simulink model "acf_force_control_simple"  (R2026b)
settings: Solver=ode4  StopTime=4  FixedStep=1.0000000000000001e-05
InitFcn:
  | acf_select_actuator(bdroot);
model workspace (MAT data in the model file):
  acfControlVersion = 'inertial-delivery-v8'
  acfImplementation = 'simple'
  acfLayoutVersion = 1
  p : object (value not decoded)
  pCompliant : object (value not decoded)
  pNearContact : object (value not decoded)
  pNoSprings : object (value not decoded)
  pRecommended : object (value not decoded)
symbols that are objects in the model workspace (value not decoded): p
undefined symbols (not defined in the file): DiscIntNeverNeededParam
(part 2 of 3)

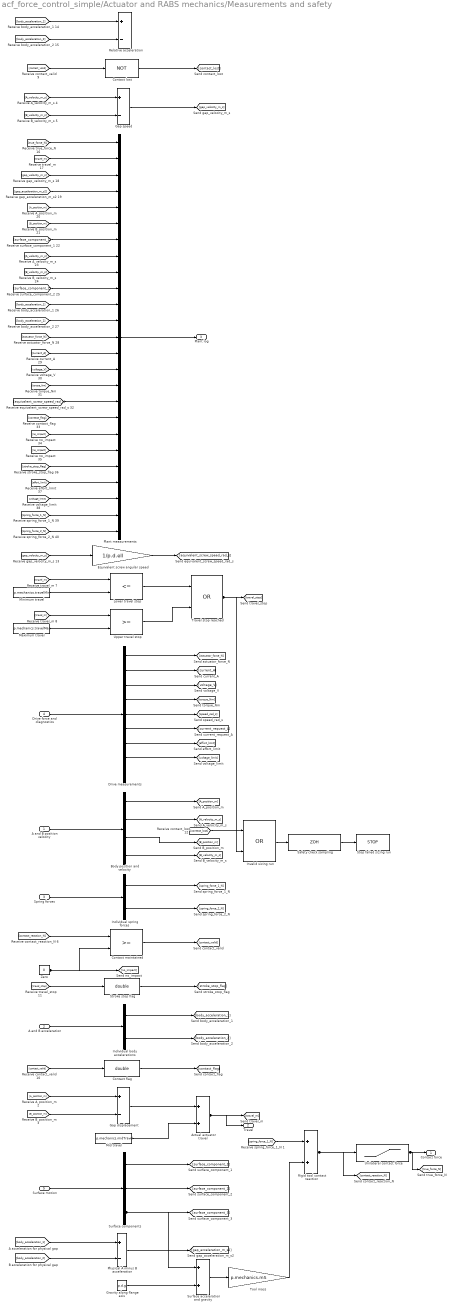
== system acf_force_control_simple/Actuator and RABS mechanics/Measurements and safety ==
  A and B position velocity : Inport
  A and B acceleration : Inport  Port=2
  Spring forces : Inport  Port=3
  Drive force and diagnostics : Inport  Port=4
  Surface motion : Inport  Port=5
  Actual actuator travel : Sum
  Body position and velocity : Demux
  Contact flag : DataTypeConversion  OutDataTypeStr=double  SaturateOnIntegerOverflow=off  RndMeth=Floor
  Contact lost : Logic  Operator=NOT  AllPortsSameDT=off  OutDataTypeStr=boolean
  Contact maintained : RelationalOperator  OutDataTypeStr=boolean  RndMeth=Simplest  InputSameDT=off
  Drive measurements : Demux  Outputs=9
  Equivalent screw angular speed : Gain  Gain=1/p.d.ell
  Gap displacement : Sum  Inputs=+-
  Gap speed : Sum  Inputs=+-
  Gravity along flange axis : Constant  Value=p.d.g
  Individual body accelerations : Demux  Outputs=2
  Individual spring forces : Demux  Outputs=2
  Invalid sizing run : Logic  Operator=OR  AllPortsSameDT=off  OutDataTypeStr=boolean
  Lower travel stop : RelationalOperator  Operator=<=  OutDataTypeStr=boolean  RndMeth=Simplest  InputSameDT=off
  Maximum travel : Constant  Value=p.mechanics.travelMax
  Mid travel : Constant  Value=p.mechanics.midTravel
  Minimum travel : Constant  Value=p.mechanics.travelMin
  Physical A minus B acceleration : Sum  Inputs=+-
  Plant measurements : Mux  Inputs=25
  Relative acceleration : Sum  Inputs=+-
  Rigid tool contact reaction : Sum
  Safety check sampling : ZeroOrderHold  SampleTime=p.sim.step
  Stop failed sizing run : Stop
  Stroke stop flag : DataTypeConversion  OutDataTypeStr=double  SaturateOnIntegerOverflow=off  RndMeth=Floor
  Surface acceleration and gravity : Sum
  Surface components : Demux  Outputs=3
  Tool mass : Gain  Gain=p.mechanics.mS
  Travel stop reached : Logic  Operator=OR  AllPortsSameDT=off  OutDataTypeStr=boolean
  Unilateral contact force : Saturate  UpperLimit=inf  LowerLimit=0
  Upper travel stop : RelationalOperator  OutDataTypeStr=boolean  RndMeth=Simplest  InputSameDT=off
  Zero : Constant  Value=0
  Contact force : Outport
  Travel : Outport  Port=2
  Plant log : Outport  Port=3
  wires:
  Tool mass/1 -> Rigid tool contact reaction/2
  Surface acceleration and gravity/1 -> Tool mass/1
  Actual actuator travel/1 -> Travel/1, [travel_m]
  [contact_lost] -> Invalid sizing run/1
  Travel stop reached/1 -> [travel_stop], Invalid sizing run/2
  Physical A minus B acceleration/1 -> [gap_acceleration_m_s2]
  Surface components/3 -> Surface acceleration and gravity/1, [surface_component_3]
  Surface components/2 -> [surface_component_2]
  Surface components/1 -> [surface_component_1]
  Mid travel/1 -> Actual actuator travel/2
  Gap displacement/1 -> Actual actuator travel/1
  Contact flag/1 -> [contact_flag]
  Individual body accelerations/2 -> [body_acceleration_2]
  Individual body accelerations/1 -> [body_acceleration_1]
  Stroke stop flag/1 -> [stroke_stop_flag]
  Rigid tool contact reaction/1 -> Unilateral contact force/1, [contact_reaction_N]
  Contact maintained/1 -> [contact_valid]
  Individual spring forces/2 -> [spring_force_2_N]
  Body position and velocity/4 -> [B_velocity_m_s]
  Drive measurements/8 -> [voltage_limit]
  Drive measurements/6 -> [current_request_A]
  [spring_force_1_N] -> Plant measurements/24
  Lower travel stop/1 -> Travel stop reached/1
  [effort_limit] -> Plant measurements/22
  Safety check sampling/1 -> Stop failed sizing run/1
  [body_acceleration_2] -> Plant measurements/12
  [stroke_stop_flag] -> Plant measurements/21
  Drive measurements/7 -> [effort_limit]
  [body_acceleration_2] -> Relative acceleration/2
  [equivalent_screw_speed_rad_s] -> Plant measurements/17
  Drive measurements/2 -> [current_A]
  [voltage_V] -> Plant measurements/15
  A and B position velocity/1 -> Body position and velocity/1
  [no_impact] -> Plant measurements/20
  [contact_flag] -> Plant measurements/18
  Body position and velocity/2 -> [A_velocity_m_s]
  [travel_stop] -> Stroke stop flag/1
  [B_velocity_m_s] -> Plant measurements/9
  [true_force_N] -> Plant measurements/1
  [no_impact] -> Plant measurements/19
  Unilateral contact force/1 -> Contact force/1, [true_force_N]
  Gap speed/1 -> [gap_velocity_m_s]
  [spring_force_2_N] -> Plant measurements/25
  [body_acceleration_1] -> Relative acceleration/1
  [B_position_m] -> Gap displacement/2
  [surface_component_1] -> Plant measurements/7
  [A_velocity_m_s] -> Plant measurements/8
  [body_acceleration_1] -> Plant measurements/11
  [surface_component_2] -> Plant measurements/10
  [travel_m] -> Lower travel stop/1
  [gap_velocity_m_s] -> Plant measurements/3
  [torque_Nm] -> Plant measurements/16
  [A_velocity_m_s] -> Gap speed/1
  Body position and velocity/3 -> [B_position_m]
  [voltage_limit] -> Plant measurements/23
  [spring_force_1_N] -> Rigid tool contact reaction/1
  [B_position_m] -> Plant measurements/6
  [travel_m] -> Plant measurements/2
  [contact_valid] -> Contact lost/1
  [B_velocity_m_s] -> Gap speed/2
  [gap_acceleration_m_s2] -> Plant measurements/4
  Zero/1 -> [no_impact], Contact maintained/2
  Maximum travel/1 -> Upper travel stop/2
  [current_A] -> Plant measurements/14
  Drive measurements/1 -> [actuator_force_N]
  [A_position_m] -> Plant measurements/5
  Minimum travel/1 -> Lower travel stop/2
  [gap_velocity_m_s] -> Equivalent screw angular speed/1
  [travel_m] -> Upper travel stop/1
  Drive force and diagnostics/1 -> Drive measurements/1
  Spring forces/1 -> Individual spring forces/1
  Invalid sizing run/1 -> Safety check sampling/1
  Gravity along flange axis/1 -> Surface acceleration and gravity/2
  [contact_reaction_N] -> Contact maintained/1
  [actuator_force_N] -> Plant measurements/13
  A and B acceleration/1 -> Individual body accelerations/1
  [contact_valid] -> Contact flag/1
  [A_position_m] -> Gap displacement/1
  Surface motion/1 -> Surface components/1
  [body_acceleration_1] -> Physical A minus B acceleration/1
  [body_acceleration_2] -> Physical A minus B acceleration/2
  Contact lost/1 -> [contact_lost]
  Plant measurements/1 -> Plant log/1
  Equivalent screw angular speed/1 -> [equivalent_screw_speed_rad_s]
  Upper travel stop/1 -> Travel stop reached/2
  Individual spring forces/1 -> [spring_force_1_N]
  Drive measurements/5 -> [speed_rad_s]
  Body position and velocity/1 -> [A_position_m]
  Drive measurements/3 -> [voltage_V]
  Drive measurements/4 -> [torque_Nm]

== system acf_force_control_simple/Actuator and RABS mechanics/R to A spring and damper ==
  A position velocity : Inport
  R position velocity : Inport  Port=2
  Rigid reaction : Inport  Port=3
  Compliant or rigid link : VariantSource  VariantControlMode=label  LabelModeActiveChoice=Rigid  VariantControls={Compliant, Rigid}
  Damping : Gain  Gain=p.mechanics.c2
  Endpoint difference : Sum  Inputs=+-
  Preload : Constant  Value=p.d.q20
  Spring and damper force : Sum  Inputs=+++
  Spring displacement and relative velocity : Demux  Outputs=2
  Stiffness : Gain  Gain=p.mechanics.k2
  Spring force : Outport
  wires:
  Compliant or rigid link/1 -> Spring force/1
  Rigid reaction/1 -> Compliant or rigid link/2
  Spring and damper force/1 -> Compliant or rigid link/1
  Preload/1 -> Spring and damper force/1
  Spring displacement and relative velocity/1 -> Stiffness/1
  Spring displacement and relative velocity/2 -> Damping/1
  Endpoint difference/1 -> Spring displacement and relative velocity/1
  Damping/1 -> Spring and damper force/3
  Stiffness/1 -> Spring and damper force/2
  R position velocity/1 -> Endpoint difference/2
  A position velocity/1 -> Endpoint difference/1

== system acf_force_control_simple/Contact force measurement/Contact force reconstruction ==
  raw_cell_error_N : Inport
  Cell error to deviation : Gain  Gain=-1
  Compensated axial reaction : Sum
  Compensated lateral reaction : Sum
  Downstream X inertia : Gain  Gain=p.sensor.distalMass_model_kg
  Downstream Z inertia : Gain  Gain=p.sensor.distalMass_model_kg
  Tared axial cell force : Bias  Bias=p.force.reference  SaturateOnIntegerOverflow=off
  axial_contact_N : Outport
  lateral_contact_N : Outport  Port=2
  tag scope: inertial_axial_contact_N=global, inertial_lateral_contact_N=global
  wires:
  Compensated lateral reaction/1 -> lateral_contact_N/1, [inertial_lateral_contact_N]
  Cell error to deviation/1 -> Tared axial cell force/1
  Compensated axial reaction/1 -> axial_contact_N/1, [inertial_axial_contact_N]
  [measured_S_acceleration_z] -> Downstream Z inertia/1
  Downstream X inertia/1 -> Compensated lateral reaction/2
  Tared axial cell force/1 -> Compensated axial reaction/1
  [measured_lateral_contact_N] -> Compensated lateral reaction/1
  Downstream Z inertia/1 -> Compensated axial reaction/2
  raw_cell_error_N/1 -> Cell error to deviation/1
  [measured_S_acceleration_x] -> Downstream X inertia/1

== system acf_force_control_simple/Contact force measurement/Head motion estimator ==
  measured_head_position_m : Inport
  Causal motion measurements : Mux  Inputs=3
  Estimated head travel : Bias  Bias=p.mechanics.midTravel+p.d.u0  SaturateOnIntegerOverflow=off
  Fresh 10 kHz position frame : ZeroOrderHold  SampleTime=p.force.sampleTime
  Fresh 10 kHz robot acceleration frame : ZeroOrderHold  SampleTime=p.force.sampleTime
  Fresh 10 kHz robot velocity frame : ZeroOrderHold  SampleTime=p.force.sampleTime
  Head gap and velocity observer : DiscreteStateSpace  A=p.d.toolMotionObserver.A  B=p.d.toolMotionObserver.B  C=p.d.toolMotionObserver.C  D=p.d.toolMotionObserver.D  InitialCondition=zeros(2,1)  SampleTime=p.force.sampleTime
  Head gap coordinate sign : Gain  Gain=-1
  Head gap displacement : Selector  InputPortWidth=2  IndexOptions=Index vector (dialog)  Indices=1  OutputSizes=1
  Head gap velocity : Selector  InputPortWidth=2  IndexOptions=Index vector (dialog)  Indices=2  OutputSizes=1
  Measured head coordinate deviation : Bias  Bias=p.d.positionMeasurementBias  SaturateOnIntegerOverflow=off
  Position common AA and EMA : DiscreteTransferFcn  Numerator=p.d.acquisition.responses.position.numerator  Denominator=p.d.acquisition.responses.position.denominator  InitialStates=(0)*p.d.acquisition.responses.position.steadyStatePerUnitInput  SampleTime=p.sensor.sampleTime
  Robot acceleration common AA and EMA : DiscreteTransferFcn  Numerator=p.d.acquisition.responses.frame.numerator  Denominator=p.d.acquisition.responses.frame.denominator  InitialStates=(0)*p.d.acquisition.responses.frame.steadyStatePerUnitInput  SampleTime=p.sensor.sampleTime
  Robot acceleration frame matching delay : Delay  DelayLength=p.d.acquisition.frameDelaySamples  InitialCondition=0  SampleTime=p.sensor.sampleTime
  Robot velocity common AA and EMA : DiscreteTransferFcn  Numerator=p.d.acquisition.responses.frame.numerator  Denominator=p.d.acquisition.responses.frame.denominator  InitialStates=(0)*p.d.acquisition.responses.frame.steadyStatePerUnitInput  SampleTime=p.sensor.sampleTime
  Robot velocity frame matching delay : Delay  DelayLength=p.d.acquisition.frameDelaySamples  InitialCondition=0  SampleTime=p.sensor.sampleTime
  head_gap_velocity_m_s : Outport
  estimated_head_travel_m : Outport  Port=2
  tag scope: inertial_head_motion_states=global, inertial_robot_acceleration_aligned=global, inertial_robot_velocity_aligned=global
  wires:
  Head gap displacement/1 -> Estimated head travel/1
  Head gap and velocity observer/1 -> [inertial_head_motion_states], Head gap velocity/1, Head gap displacement/1
  Causal motion measurements/1 -> Head gap and velocity observer/1
  Fresh 10 kHz robot acceleration frame/1 -> Causal motion measurements/2, [inertial_robot_acceleration_aligned]
  measured_head_position_m/1 -> Measured head coordinate deviation/1
  Measured head coordinate deviation/1 -> Head gap coordinate sign/1
  Robot velocity frame matching delay/1 -> Fresh 10 kHz robot velocity frame/1
  Robot velocity common AA and EMA/1 -> Robot velocity frame matching delay/1
  Robot acceleration common AA and EMA/1 -> Robot acceleration frame matching delay/1
  Estimated head travel/1 -> estimated_head_travel_m/1
  Head gap coordinate sign/1 -> Position common AA and EMA/1
  Robot acceleration frame matching delay/1 -> Fresh 10 kHz robot acceleration frame/1
  Position common AA and EMA/1 -> Fresh 10 kHz position frame/1
  Fresh 10 kHz robot velocity frame/1 -> [inertial_robot_velocity_aligned]
  [command_based_robot_velocity] -> Robot velocity common AA and EMA/1
  [command_based_robot_acceleration] -> Robot acceleration common AA and EMA/1
  Fresh 10 kHz position frame/1 -> Causal motion measurements/1
  Head gap velocity/1 -> head_gap_velocity_m_s/1
  [measured_S_acceleration_z] -> Causal motion measurements/3

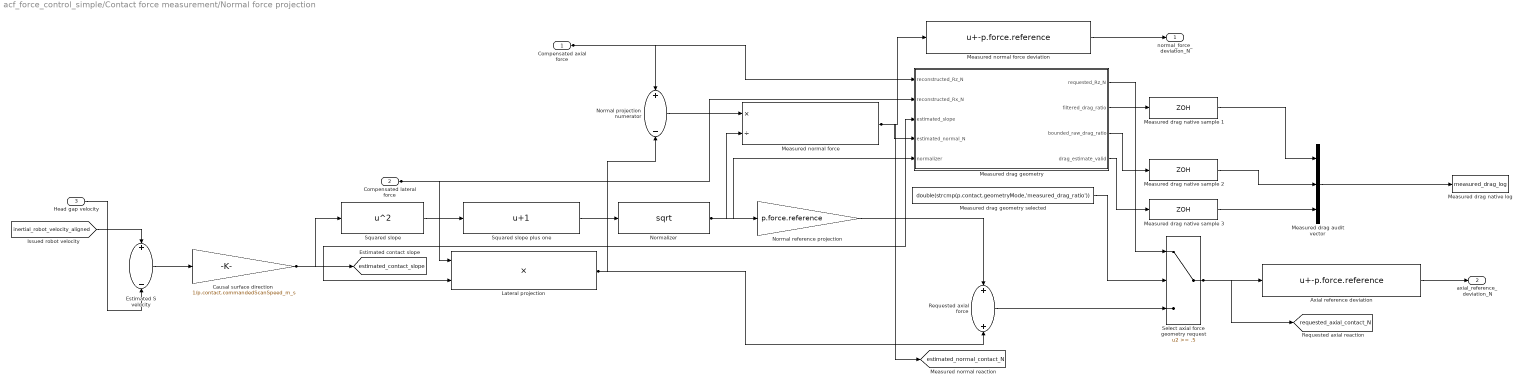
== system acf_force_control_simple/Contact force measurement/Normal force projection ==
  Compensated axial force : Inport
  Compensated lateral force : Inport  Port=2
  Head gap velocity : Inport  Port=3
  Axial reference deviation : Bias  Bias=-p.force.reference  SaturateOnIntegerOverflow=off
  Causal surface direction : Gain  Gain=1/p.contact.commandedScanSpeed_m_s
  Estimated S velocity : Sum  Inputs=+-
  Lateral projection : Product  Inputs=**
  Measured drag audit vector : Mux  Inputs=3
  Measured drag geometry : Subsystem
  Measured drag geometry selected : Constant  Value=double(strcmp(p.contact.geometryMode,'measured_drag_ratio'))
  Measured drag native log : ToWorkspace  VariableName=measured_drag_log  SaveFormat=Timeseries  SampleTime=-1
  Measured drag native sample 1 : ZeroOrderHold  SampleTime=p.sim.step
  Measured drag native sample 2 : ZeroOrderHold  SampleTime=p.sim.step
  Measured drag native sample 3 : ZeroOrderHold  SampleTime=p.sim.step
  Measured normal force : Product  Inputs=*/
  Measured normal force deviation : Bias  Bias=-p.force.reference  SaturateOnIntegerOverflow=off
  Normal projection numerator : Sum  Inputs=+-
  Normal reference projection : Gain  Gain=p.force.reference
  Normalizer : Math  Operator=sqrt
  Requested axial force : Sum
  Select axial force geometry request : Switch  Threshold=.5  SaturateOnIntegerOverflow=off  InputSameDT=off
  Squared slope : Math  Operator=square
  Squared slope plus one : Bias  Bias=1  SaturateOnIntegerOverflow=off
  normal_force_deviation_N : Outport
  axial_reference_deviation_N : Outport  Port=2
  tag scope: estimated_contact_slope=global, estimated_normal_contact_N=global, requested_axial_contact_N=global
  wires:
  Measured drag audit vector/1 -> Measured drag native log/1
  Measured drag native sample 2/1 -> Measured drag audit vector/2
  Axial reference deviation/1 -> axial_reference_deviation_N/1
  Requested axial force/1 -> Select axial force geometry request/3
  Measured drag geometry/4(drag_estimate_valid) -> Measured drag native sample 3/1
  Measured drag geometry/3(bounded_raw_drag_ratio) -> Measured drag native sample 2/1
  Measured drag geometry/2(filtered_drag_ratio) -> Measured drag native sample 1/1
  Measured drag geometry/1(requested_Rz_N) -> Select axial force geometry request/1
  Measured normal force deviation/1 -> normal_force_deviation_N/1
  Head gap velocity/1 -> Estimated S velocity/2
  [inertial_robot_velocity_aligned] -> Estimated S velocity/1
  Squared slope/1 -> Squared slope plus one/1
  Normalizer/1 -> Measured normal force/2, Normal reference projection/1, Measured drag geometry/5(normalizer)
  Causal surface direction/1 -> Squared slope/1, [estimated_contact_slope], Lateral projection/2, Measured drag geometry/3(estimated_slope)
  Measured drag geometry selected/1 -> Select axial force geometry request/2
  Normal projection numerator/1 -> Measured normal force/1
  Measured drag native sample 1/1 -> Measured drag audit vector/1
  Compensated lateral force/1 -> Lateral projection/1, Measured drag geometry/2(reconstructed_Rx_N)
  Compensated axial force/1 -> Normal projection numerator/1, Measured drag geometry/1(reconstructed_Rz_N)
  Select axial force geometry request/1 -> Axial reference deviation/1, [requested_axial_contact_N]
  Squared slope plus one/1 -> Normalizer/1
  Estimated S velocity/1 -> Causal surface direction/1
  Measured normal force/1 -> Measured normal force deviation/1, [estimated_normal_contact_N], Measured drag geometry/4(estimated_normal_N)
  Lateral projection/1 -> Normal projection numerator/2, Requested axial force/2
  Measured drag native sample 3/1 -> Measured drag audit vector/3
  Normal reference projection/1 -> Requested axial force/1

== system acf_force_control_simple/Force controller/Coil PI and PID ==
  error_N : Inport
  measured_travel_m : Inport  Port=2
  Current limits : Saturate  UpperLimit=p.coil.peakCurrent  LowerLimit=-p.coil.peakCurrent
  Current saturation error : Sum  Inputs=+-
  Flat holding current : Constant  Value=p.d.coilHoldingCurrentCommand_A
  Integral anti windup : Gain  Gain=-p.force.antiWindupRate/p.inertial.forceKi
  Lower spring inverse feedforward : Subsystem
  Measured motion feedforward : Subsystem
  Normal force PI and PID : Subsystem
  Optional structural-mode current notch : DiscreteTransferFcn  Numerator=p.d.currentNotch.numerator  Denominator=p.d.currentNotch.denominator  InitialStates=p.d.currentNotch.initialStates  SampleTime=p.force.sampleTime
  PI PID and feedforward current : Sum  Inputs=++++++
  command : Outport
  estimated_travel_m : Outport  Port=2
  estimated_force_error_N : Outport  Port=3
  wires:
  Current saturation error/1 -> Integral anti windup/1
  Current limits/1 -> command/1, Current saturation error/1
  PI PID and feedforward current/1 -> Optional structural-mode current notch/1
  Measured motion feedforward/3(friction_current_A) -> PI PID and feedforward current/5
  Measured motion feedforward/1(acceleration_current_A) -> PI PID and feedforward current/3
  Flat holding current/1 -> PI PID and feedforward current/1
  Optional structural-mode current notch/1 -> Current limits/1, Current saturation error/2
  Lower spring inverse feedforward/1(extra_current_A) -> PI PID and feedforward current/6
  Measured motion feedforward/2(geometry_current_A) -> PI PID and feedforward current/4
  Normal force PI and PID/1(feedback_current_A) -> PI PID and feedforward current/2
  error_N/1 -> Normal force PI and PID/1(error_N), estimated_force_error_N/1
  Integral anti windup/1 -> Normal force PI and PID/2(anti_windup)
  measured_travel_m/1 -> estimated_travel_m/1

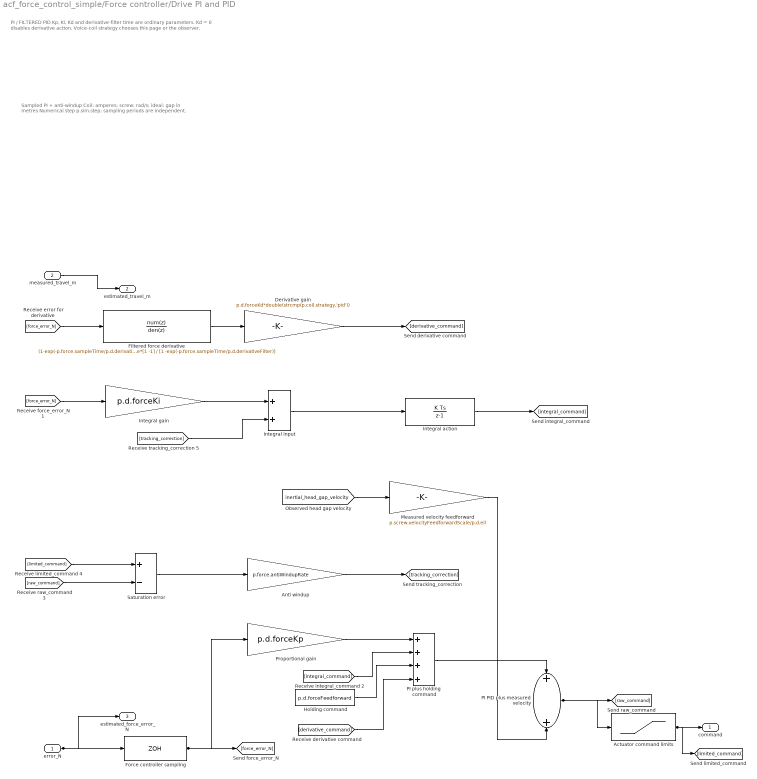
== system acf_force_control_simple/Force controller/Drive PI and PID ==
  note: Sampled PI + anti-windup
      | Coil: amperes; screw: rad/s; ideal: gap in metres
      | Numerical step p.sim.step; sampling periods are independent.
  note: PI / FILTERED PID
      | Kp, Ki, Kd and derivative-filter time are ordinary parameters.
      | Kd = 0 disables derivative action. Voice-coil strategy chooses this page or the observer.
  error_N : Inport
  measured_travel_m : Inport  Port=2
  Actuator command limits : Saturate  UpperLimit=p.d.commandMax  LowerLimit=p.d.commandMin
  Anti windup : Gain  Gain=p.force.antiWindupRate
  Derivative gain : Gain  Gain=p.d.forceKd*double(strcmp(p.coil.strategy,'pid'))
  Filtered force derivative : DiscreteTransferFcn  Numerator=(1-exp(-p.force.sampleTime/p.d.derivativeFilter))/p.force.sampleTime*[1 -1]  Denominator=[1 -exp(-p.force.sampleTime/p.d.derivativeFilter)]  SampleTime=p.force.sampleTime
  Force controller sampling : ZeroOrderHold  SampleTime=p.force.sampleTime
  Holding command : Constant  Value=p.d.forceFeedforward
  Integral action : DiscreteIntegrator  SampleTime=p.force.sampleTime  ICPrevOutput=DiscIntNeverNeededParam  ICPrevScaledInput=DiscIntNeverNeededParam
  Integral gain : Gain  Gain=p.d.forceKi
  Integral input : Sum
  Measured velocity feedforward : Gain  Gain=p.screw.velocityFeedforwardScale/p.d.ell
  PI PID plus measured velocity : Sum
  PI plus holding command : Sum  Inputs=++++
  Proportional gain : Gain  Gain=p.d.forceKp
  Saturation error : Sum  Inputs=+-
  command : Outport
  estimated_travel_m : Outport  Port=2
  estimated_force_error_N : Outport  Port=3
  wires:
  PI plus holding command/1 -> PI PID plus measured velocity/1
  [derivative_command] -> PI plus holding command/4
  Holding command/1 -> PI plus holding command/3
  [integral_command] -> PI plus holding command/2
  Proportional gain/1 -> PI plus holding command/1
  Anti windup/1 -> [tracking_correction]
  [inertial_head_gap_velocity] -> Measured velocity feedforward/1
  Filtered force derivative/1 -> Derivative gain/1
  [tracking_correction] -> Integral input/2
  Derivative gain/1 -> [derivative_command]
  Actuator command limits/1 -> [limited_command], command/1
  [force_error_N] -> Integral gain/1
  PI PID plus measured velocity/1 -> Actuator command limits/1, [raw_command]
  Integral action/1 -> [integral_command]
  measured_travel_m/1 -> estimated_travel_m/1
  [limited_command] -> Saturation error/1
  Saturation error/1 -> Anti windup/1
  [raw_command] -> Saturation error/2
  [force_error_N] -> Filtered force derivative/1
  error_N/1 -> estimated_force_error_N/1, Force controller sampling/1
  Integral gain/1 -> Integral input/1
  Force controller sampling/1 -> Proportional gain/1, [force_error_N]
  Measured velocity feedforward/1 -> PI PID plus measured velocity/2
  Integral input/1 -> Integral action/1

== system acf_force_control_simple/Force controller/Screw normal PI and PID ==
  error_N : Inport
  measured_travel_m : Inport  Port=2
  Current limits : Saturate  UpperLimit=p.screw.peakCurrent  LowerLimit=-p.screw.peakCurrent
  Current saturation error : Sum  Inputs=+-
  Flat holding current : Constant  Value=p.d.screwHoldingCurrentCommand_A
  Integral anti windup : Gain  Gain=-p.force.antiWindupRate/p.screw.currentForceKi
  Lower spring inverse feedforward : Subsystem
  Measured motion feedforward : Subsystem
  Normal force PI and PID : Subsystem
  Optional structural-mode current notch : DiscreteTransferFcn  Numerator=p.d.screwCurrentNotch.numerator  Denominator=p.d.screwCurrentNotch.denominator  InitialStates=p.d.screwCurrentNotch.initialStates  SampleTime=p.force.sampleTime
  PI PID and feedforward current : Sum  Inputs=++++++
  command : Outport
  estimated_travel_m : Outport  Port=2
  estimated_force_error_N : Outport  Port=3
  wires:
  Optional structural-mode current notch/1 -> Current limits/1, Current saturation error/2
  PI PID and feedforward current/1 -> Optional structural-mode current notch/1
  Current limits/1 -> command/1, Current saturation error/1
  Lower spring inverse feedforward/1(extra_current_A) -> PI PID and feedforward current/6
  Current saturation error/1 -> Integral anti windup/1
  Measured motion feedforward/3(friction_current_A) -> PI PID and feedforward current/5
  Measured motion feedforward/2(geometry_current_A) -> PI PID and feedforward current/4
  Integral anti windup/1 -> Normal force PI and PID/2(anti_windup)
  Measured motion feedforward/1(acceleration_current_A) -> PI PID and feedforward current/3
  Flat holding current/1 -> PI PID and feedforward current/1
  Normal force PI and PID/1(feedback_current_A) -> PI PID and feedforward current/2
  error_N/1 -> estimated_force_error_N/1, Normal force PI and PID/1(error_N)
  measured_travel_m/1 -> estimated_travel_m/1

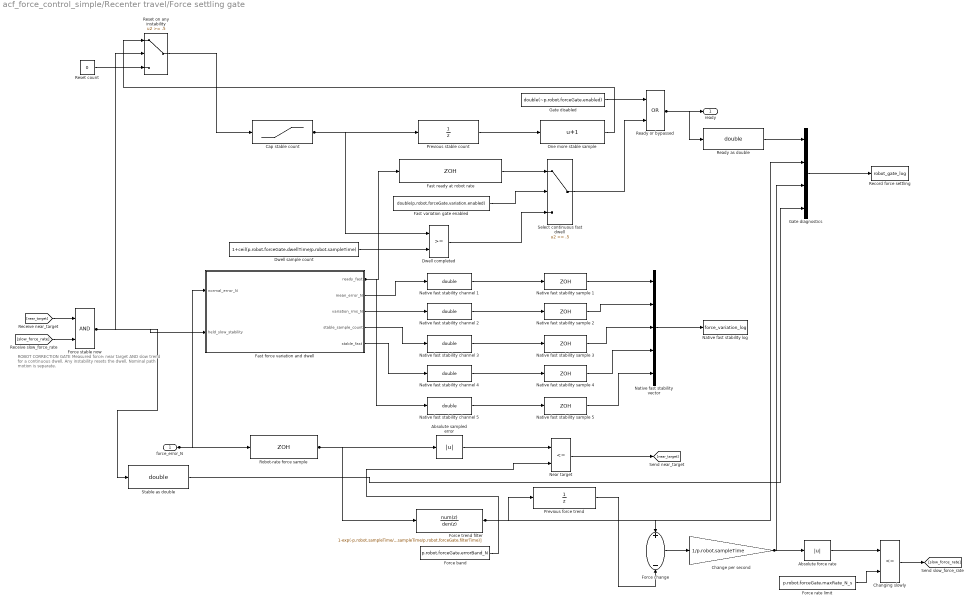
== system acf_force_control_simple/Recenter travel/Force settling gate ==
  note: ROBOT CORRECTION GATE
      | Measured force: near target AND slow trend for a continuous dwell.
      | Any instability resets the dwell. Nominal path motion is separate.
  force_error_N : Inport
  Absolute force rate : Abs  SaturateOnIntegerOverflow=off
  Absolute sampled error : Abs  SaturateOnIntegerOverflow=off
  Cap stable count : Saturate  UpperLimit=1+ceil(p.robot.forceGate.dwellTime/p.robot.sampleTime)  LowerLimit=0
  Change per second : Gain  Gain=1/p.robot.sampleTime
  Changing slowly : RelationalOperator  Operator=<=  OutDataTypeStr=boolean  RndMeth=Simplest  InputSameDT=off
  Dwell completed : RelationalOperator  OutDataTypeStr=boolean  RndMeth=Simplest  InputSameDT=off
  Dwell sample count : Constant  Value=1+ceil(p.robot.forceGate.dwellTime/p.robot.sampleTime)
  Fast force variation and dwell : Subsystem
  Fast ready at robot rate : ZeroOrderHold  SampleTime=p.robot.sampleTime
  Fast variation gate enabled : Constant  Value=double(p.robot.forceGate.variation.enabled)
  Force band : Constant  Value=p.robot.forceGate.errorBand_N
  Force change : Sum  Inputs=+-
  Force rate limit : Constant  Value=p.robot.forceGate.maxRate_N_s
  Force stable now : Logic  AllPortsSameDT=off  OutDataTypeStr=boolean
  Force trend filter : DiscreteTransferFcn  Numerator=1-exp(-p.robot.sampleTime/p.robot.forceGate.filterTime)  Denominator=[1 -exp(-p.robot.sampleTime/p.robot.forceGate.filterTime)]  SampleTime=p.robot.sampleTime
  Gate diagnostics : Mux
  Gate disabled : Constant  Value=double(~p.robot.forceGate.enabled)
  Native fast stability channel {1..5} (5 alike) : DataTypeConversion  OutDataTypeStr=double  SaturateOnIntegerOverflow=off  RndMeth=Floor
  Native fast stability log : ToWorkspace  VariableName=force_variation_log  SaveFormat=Timeseries  SampleTime=-1
  Native fast stability sample {1..5} (5 alike) : ZeroOrderHold  SampleTime=p.sim.step
  Native fast stability vector : Mux  Inputs=5
  Near target : RelationalOperator  Operator=<=  OutDataTypeStr=boolean  RndMeth=Simplest  InputSameDT=off
  One more stable sample : Bias  Bias=1  SaturateOnIntegerOverflow=off
  Previous force trend : UnitDelay  SampleTime=p.robot.sampleTime
  Previous stable count : UnitDelay  SampleTime=p.robot.sampleTime
  Ready as double : DataTypeConversion  OutDataTypeStr=double  SaturateOnIntegerOverflow=off  RndMeth=Floor
  Ready or bypassed : Logic  Operator=OR  AllPortsSameDT=off  OutDataTypeStr=boolean
  Record force settling : ToWorkspace  VariableName=robot_gate_log  SaveFormat=Timeseries  SampleTime=p.robot.sampleTime
  Reset count : Constant  Value=0
  Reset on any instability : Switch  Threshold=.5  SaturateOnIntegerOverflow=off  InputSameDT=off
  Robot-rate force sample : ZeroOrderHold  SampleTime=p.robot.sampleTime
  Select continuous fast dwell : Switch  Threshold=.5  SaturateOnIntegerOverflow=off  InputSameDT=off
  Stable as double : DataTypeConversion  OutDataTypeStr=double  SaturateOnIntegerOverflow=off  RndMeth=Floor
  ready : Outport
  wires:
  Force rate limit/1 -> Changing slowly/2
  Changing slowly/1 -> [slow_force_rate]
  Gate diagnostics/1 -> Record force settling/1
  Native fast stability vector/1 -> Native fast stability log/1
  Ready as double/1 -> Gate diagnostics/1
  Previous force trend/1 -> Force change/2
  Native fast stability sample 4/1 -> Native fast stability vector/4
  Native fast stability sample 1/1 -> Native fast stability vector/1
  Select continuous fast dwell/1 -> Ready or bypassed/2
  Fast force variation and dwell/1(ready_fast) -> Native fast stability channel 5/1, Fast ready at robot rate/1
  [slow_force_rate] -> Force stable now/2
  Force change/1 -> Change per second/1
  Native fast stability channel 4/1 -> Native fast stability sample 4/1
  Dwell sample count/1 -> Dwell completed/2
  Absolute force rate/1 -> Changing slowly/1
  Ready or bypassed/1 -> Ready as double/1, ready/1
  Reset on any instability/1 -> Cap stable count/1
  Native fast stability sample 2/1 -> Native fast stability vector/2
  Cap stable count/1 -> Dwell completed/1, Previous stable count/1
  Stable as double/1 -> Gate diagnostics/4
  Force trend filter/1 -> Previous force trend/1, Force change/1, Gate diagnostics/2
  Gate disabled/1 -> Ready or bypassed/1
  Fast force variation and dwell/3(variation_rms_N) -> Native fast stability channel 2/1
  [near_target] -> Force stable now/1
  Change per second/1 -> Gate diagnostics/3, Absolute force rate/1
  Near target/1 -> [near_target]
  Native fast stability sample 3/1 -> Native fast stability vector/3
  Fast force variation and dwell/5(stable_fast) -> Native fast stability channel 4/1
  Fast force variation and dwell/4(stable_sample_count) -> Native fast stability channel 3/1
  Force stable now/1 -> Stable as double/1, Reset on any instability/2, Fast force variation and dwell/2(held_slow_stability)
  Previous stable count/1 -> One more stable sample/1
  Fast variation gate enabled/1 -> Select continuous fast dwell/2
  Fast ready at robot rate/1 -> Select continuous fast dwell/1
  Dwell completed/1 -> Select continuous fast dwell/3
  Native fast stability channel 3/1 -> Native fast stability sample 3/1
  Native fast stability channel 1/1 -> Native fast stability sample 1/1
  force_error_N/1 -> Fast force variation and dwell/1(normal_error_N), Robot-rate force sample/1
  Native fast stability channel 2/1 -> Native fast stability sample 2/1
  Native fast stability channel 5/1 -> Native fast stability sample 5/1
  Reset count/1 -> Reset on any instability/3
  Robot-rate force sample/1 -> Force trend filter/1, Absolute sampled error/1
  Force band/1 -> Near target/2
  Native fast stability sample 5/1 -> Native fast stability vector/5
  Fast force variation and dwell/2(mean_error_N) -> Native fast stability channel 1/1
  Absolute sampled error/1 -> Near target/1
  One more stable sample/1 -> Reset on any instability/1

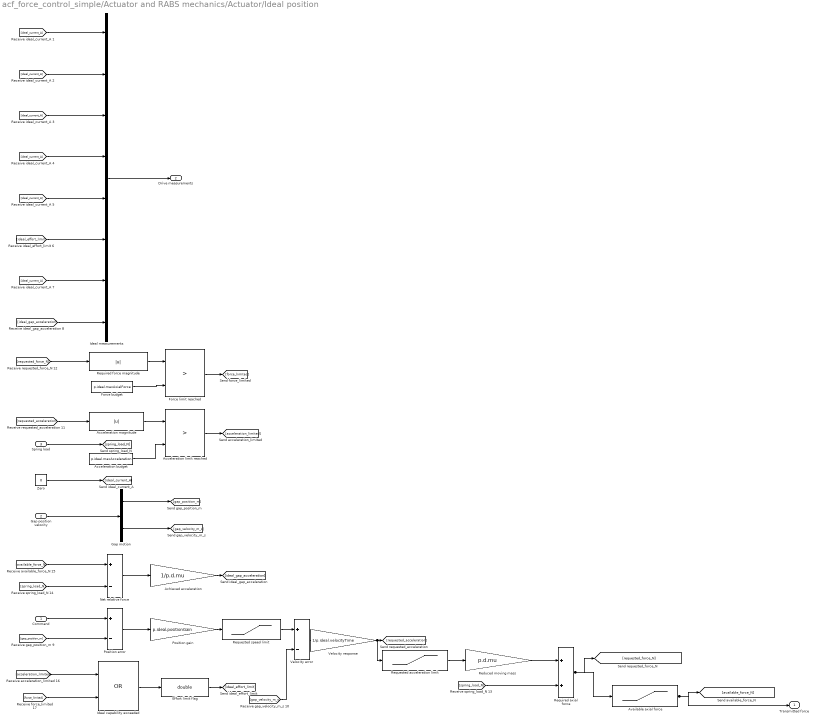
== system acf_force_control_simple/Actuator and RABS mechanics/Actuator/Ideal position ==
  Command : Inport
  Gap position velocity : Inport  Port=2
  Spring load : Inport  Port=3
  Acceleration budget : Constant  Value=p.ideal.maxAcceleration
  Acceleration limit reached : RelationalOperator  Operator=>  OutDataTypeStr=boolean  RndMeth=Simplest  InputSameDT=off
  Acceleration magnitude : Abs  SaturateOnIntegerOverflow=off
  Achieved acceleration : Gain  Gain=1/p.d.mu
  Available axial force : Saturate  UpperLimit=p.ideal.maxAxialForce  LowerLimit=-p.ideal.maxAxialForce
  Effort limit flag : DataTypeConversion  OutDataTypeStr=double  SaturateOnIntegerOverflow=off  RndMeth=Floor
  Force budget : Constant  Value=p.ideal.maxAxialForce
  Force limit reached : RelationalOperator  Operator=>  OutDataTypeStr=boolean  RndMeth=Simplest  InputSameDT=off
  Gap motion : Demux  Outputs=2
  Ideal capability exceeded : Logic  Operator=OR  AllPortsSameDT=off  OutDataTypeStr=boolean
  Ideal measurements : Mux  Inputs=8
  Net relative force : Sum  Inputs=+-
  Position error : Sum  Inputs=+-
  Position gain : Gain  Gain=p.ideal.positionGain
  Reduced moving mass : Gain  Gain=p.d.mu
  Requested acceleration limit : Saturate  UpperLimit=p.ideal.maxAcceleration  LowerLimit=-p.ideal.maxAcceleration
  Requested speed limit : Saturate  UpperLimit=p.ideal.maxSpeed  LowerLimit=-p.ideal.maxSpeed
  Required axial force : Sum
  Required force magnitude : Abs  SaturateOnIntegerOverflow=off
  Velocity error : Sum  Inputs=+-
  Velocity response : Gain  Gain=1/p.ideal.velocityTime
  Zero : Constant  Value=0
  Transmitted force : Outport
  Drive measurements : Outport  Port=2
  wires:
  Requested acceleration limit/1 -> Reduced moving mass/1
  Required axial force/1 -> [requested_force_N], Available axial force/1
  Velocity response/1 -> [requested_acceleration], Requested acceleration limit/1
  [gap_velocity_m_s] -> Velocity error/2
  Requested speed limit/1 -> Velocity error/1
  Effort limit flag/1 -> [ideal_effort_limit]
  Position gain/1 -> Requested speed limit/1
  Achieved acceleration/1 -> [ideal_gap_acceleration]
  Acceleration limit reached/1 -> [acceleration_limited]
  Required force magnitude/1 -> Force limit reached/1
  [ideal_gap_acceleration] -> Ideal measurements/8
  [ideal_current_A] -> Ideal measurements/7
  [ideal_current_A] -> Ideal measurements/3
  [ideal_current_A] -> Ideal measurements/5
  [ideal_current_A] -> Ideal measurements/4
  [spring_load_N] -> Net relative force/2
  Ideal capability exceeded/1 -> Effort limit flag/1
  [gap_position_m] -> Position error/2
  Command/1 -> Position error/1
  Acceleration budget/1 -> Acceleration limit reached/2
  Zero/1 -> [ideal_current_A]
  Available axial force/1 -> Transmitted force/1, [available_force_N]
  [requested_force_N] -> Required force magnitude/1
  [ideal_current_A] -> Ideal measurements/2
  Force limit reached/1 -> [force_limited]
  Gap position velocity/1 -> Gap motion/1
  Spring load/1 -> [spring_load_N]
  [ideal_current_A] -> Ideal measurements/1
  Reduced moving mass/1 -> Required axial force/1
  Velocity error/1 -> Velocity response/1
  [available_force_N] -> Net relative force/1
  Ideal measurements/1 -> Drive measurements/1
  [acceleration_limited] -> Ideal capability exceeded/1
  [ideal_effort_limit] -> Ideal measurements/6
  [force_limited] -> Ideal capability exceeded/2
  [spring_load_N] -> Required axial force/2
  Force budget/1 -> Force limit reached/2
  Position error/1 -> Position gain/1
  Acceleration magnitude/1 -> Acceleration limit reached/1
  Gap motion/1 -> [gap_position_m]
  [requested_acceleration] -> Acceleration magnitude/1
  Gap motion/2 -> [gap_velocity_m_s]
  Net relative force/1 -> Achieved acceleration/1

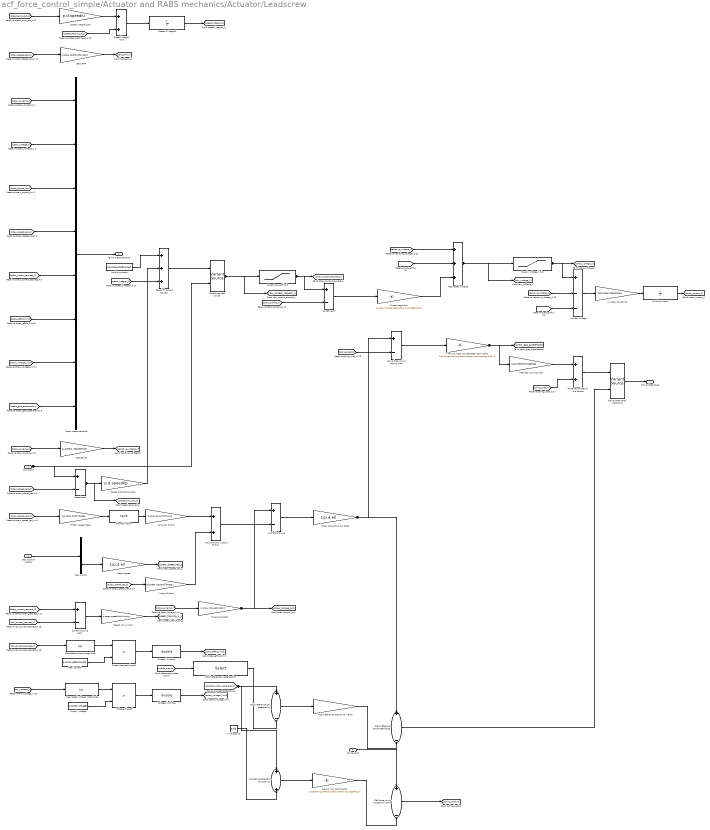
== system acf_force_control_simple/Actuator and RABS mechanics/Actuator/Leadscrew ==
  Command : Inport
  Gap position velocity : Inport  Port=2
  Spring load : Inport  Port=3
  Available torque : Sum  Inputs=+-
  Axial gravity : Constant  Value=p.d.g
  Back EMF : Gain  Gain=p.screw.backEmfConstant
  Cell force minus imposed B inertia : Sum  Inputs=+-
  Coulomb and viscous friction : Sum
  Coulomb friction : Gain  Gain=p.screw.coulombTorque
  Current clipping error : Sum  Inputs=+-
  Current error : Sum  Inputs=+-
  Current limit flag : DataTypeConversion  OutDataTypeStr=double  SaturateOnIntegerOverflow=off  RndMeth=Floor
  Current regulator : Gain  Gain=p.screw.inductance/p.screw.currentResponse
  Current request clipped : RelationalOperator  Operator=>  OutDataTypeStr=boolean  RndMeth=Simplest  InputSameDT=off
  Current request limit : Saturate  UpperLimit=p.screw.peakCurrent  LowerLimit=-p.screw.peakCurrent
  Current request source : VariantSource  VariantControlMode=label  LabelModeActiveChoice=Speed loop  VariantControls={Speed loop, Current command}
  Drive force minus spring load : Sum  Inputs=+-
  Force transmitted to the bodies : Sum
  Friction speed scale : Gain  Gain=1/p.screw.frictionSpeed
  Gap motion : Demux  Outputs=2
  Holding current : Constant  Value=p.d.screwHoldCurrent
  Imposed acceleration plus gravity : Sum
  Inductor voltage : Sum  Inputs=+--
  Inverse inductance : Gain  Gain=1/p.screw.inductance
  Moving mass and reflected rotor inertia : Gain  Gain=1/(p.d.screwMovingMass+p.screw.rotorInertia/p.d.ell^2)
  Peak current : Constant  Value=p.screw.peakCurrent
  Reduced moving mass : Gain  Gain=p.d.screwMovingMass
  Requested current magnitude : Abs  SaturateOnIntegerOverflow=off
  Requested voltage : Sum  Inputs=+++
  Requested voltage magnitude : Abs  SaturateOnIntegerOverflow=off
  Resistance : Gain  Gain=p.screw.resistance
  Rigid reference S acceleration : Selector  InputPortWidth=3  IndexOptions=Index vector (dialog)  Indices=3  OutputSizes=1
  Rigid reference gap acceleration : Sum  Inputs=+-
  Rigid reference rotor axial inertia : Gain  Gain=p.screw.rotorInertia/p.d.ell^2
  Rigid reference transmitted force : Sum  Inputs=+-
  Rigid-A moving B inertia : Gain  Gain=p.mechanics.mB*double(p.mechanics.upperRigid)
  Screw measurements : Mux  Inputs=8
  Screw speed : Gain  Gain=1/p.d.ell
  Screw torque to axial force : Gain  Gain=1/p.d.ell
  Smooth friction : Trigonometry  Operator=tanh
  Speed PI current request : Sum  Inputs=+++
  Speed PI integral : Integrator
  Speed anti windup : Gain  Gain=p.screw.speedAntiWindup
  Speed error : Sum  Inputs=+-
  Speed integral gain : Gain  Gain=p.d.speedKi
  Speed integral input : Sum
  Speed proportional gain : Gain  Gain=p.d.speedKp
  Supply voltage : Constant  Value=p.screw.voltage
  Supply voltage limits : Saturate  UpperLimit=p.screw.voltage  LowerLimit=-p.screw.voltage
  Torque constant : Gain  Gain=p.screw.torqueConstant
  Transmitted force mechanics : VariantSource  VariantControlMode=label  LabelModeActiveChoice=Finite B-S cell  VariantControls={Finite B-S cell, Rigid B-S reference}
  Viscous friction : Gain  Gain=p.screw.viscousTorque
  Voltage clipped : RelationalOperator  Operator=>  OutDataTypeStr=boolean  RndMeth=Simplest  InputSameDT=off
  Voltage limit flag : DataTypeConversion  OutDataTypeStr=double  SaturateOnIntegerOverflow=off  RndMeth=Floor
  Winding current : Integrator  InitialCondition=p.d.screwHoldCurrent
  Transmitted force : Outport
  Drive measurements : Outport  Port=2
  wires:
  Transmitted force mechanics/1 -> Transmitted force/1
  Inverse inductance/1 -> Winding current/1
  Force transmitted to the bodies/1 -> Transmitted force mechanics/1
  [spring_load_N] -> Force transmitted to the bodies/2
  Reduced moving mass/1 -> Force transmitted to the bodies/1
  Supply voltage limits/1 -> Inductor voltage/1, [screw_voltage_V]
  Requested voltage/1 -> [raw_voltage_V], Supply voltage limits/1
  Rigid reference transmitted force/1 -> Transmitted force mechanics/2
  Drive force minus spring load/1 -> Moving mass and reflected rotor inertia/1
  Current regulator/1 -> Requested voltage/3
  [back_emf_V] -> Requested voltage/2
  [resistive_voltage_V] -> Inductor voltage/2
  [resistive_voltage_V] -> Requested voltage/1
  Rigid-A moving B inertia/1 -> Cell force minus imposed B inertia/2
  [back_emf_V] -> Inductor voltage/3
  Spring load/1 -> Cell force minus imposed B inertia/1
  Rigid reference rotor axial inertia/1 -> Rigid reference transmitted force/2
  Screw torque to axial force/1 -> Drive force minus spring load/1, Rigid reference transmitted force/1
  Current error/1 -> Current regulator/1
  Rigid reference gap acceleration/1 -> Rigid reference rotor axial inertia/1
  Requested current magnitude/1 -> Current request clipped/1
  Current clipping error/1 -> Speed anti windup/1
  Speed integral gain/1 -> Speed integral input/1
  [raw_current_request_A] -> Current clipping error/2
  Current limit flag/1 -> [screw_effort_limit]
  Gap motion/2 -> Screw speed/1
  [screw_current_request_A] -> Current clipping error/1
  Friction speed scale/1 -> Smooth friction/1
  [raw_voltage_V] -> Requested voltage magnitude/1
  Peak current/1 -> Current request clipped/2
  Cell force minus imposed B inertia/1 -> [spring_load_N]
  Gap position velocity/1 -> Gap motion/1
  Command/1 -> Speed error/1, Current request source/2
  Moving mass and reflected rotor inertia/1 -> Reduced moving mass/1, [screw_gap_acceleration]
  [screw_gap_acceleration] -> Screw measurements/8
  [screw_current_A] -> Current error/2
  Back EMF/1 -> [back_emf_V]
  [raw_current_request_A] -> Requested current magnitude/1
  Current request source/1 -> [raw_current_request_A], Current request limit/1
  [surface_motion] -> Rigid reference S acceleration/1
  [screw_torque_Nm] -> Screw measurements/3
  [spring_load_N] -> Drive force minus spring load/2
  [screw_speed_rad_s] -> Viscous friction/1
  Inductor voltage/1 -> Inverse inductance/1
  [screw_speed_rad_s] -> Screw measurements/4
  [screw_current_A] -> Resistance/1
  Voltage limit flag/1 -> [screw_voltage_limit]
  [speed_tracking_A_s] -> Speed integral input/2
  [screw_speed_rad_s] -> Friction speed scale/1
  [screw_speed_rad_s] -> Back EMF/1
  Winding current/1 -> [screw_current_A]
  Requested voltage magnitude/1 -> Voltage clipped/1
  Rigid reference S acceleration/1 -> Rigid reference gap acceleration/2
  [screw_effort_limit] -> Screw measurements/6
  Screw measurements/1 -> Drive measurements/1
  [screw_voltage_limit] -> Screw measurements/7
  [screw_speed_rad_s] -> Speed error/2
  Imposed acceleration plus gravity/1 -> Rigid-A moving B inertia/1
  Supply voltage/1 -> Voltage clipped/2
  Resistance/1 -> [resistive_voltage_V]
  Speed PI current request/1 -> Current request source/1
  Axial gravity/1 -> Imposed acceleration plus gravity/2
  Current request limit/1 -> Current error/1, [screw_current_request_A]
  Speed integral input/1 -> Speed PI integral/1
  [screw_current_request_A] -> Screw measurements/5
  Speed anti windup/1 -> [speed_tracking_A_s]
  [screw_voltage_V] -> Screw measurements/2
  [robot_boundary_acceleration] -> Rigid reference gap acceleration/1, Imposed acceleration plus gravity/1
  Holding current/1 -> Speed PI current request/1
  [speed_integral_A] -> Speed PI current request/3
  Speed proportional gain/1 -> Speed PI current request/2
  Smooth friction/1 -> Coulomb friction/1
  Coulomb friction/1 -> Coulomb and viscous friction/1
  Voltage clipped/1 -> Voltage limit flag/1
  [speed_error_rad_s] -> Speed integral gain/1
  Torque constant/1 -> Available torque/1, [screw_torque_Nm]
  Speed PI integral/1 -> [speed_integral_A]
  Speed error/1 -> [speed_error_rad_s], Speed proportional gain/1
  Viscous friction/1 -> Coulomb and viscous friction/2
  [screw_current_A] -> Screw measurements/1
  Screw speed/1 -> [screw_speed_rad_s]
  Current request clipped/1 -> Current limit flag/1
  [screw_current_A] -> Torque constant/1
  Coulomb and viscous friction/1 -> Available torque/2
  Available torque/1 -> Screw torque to axial force/1

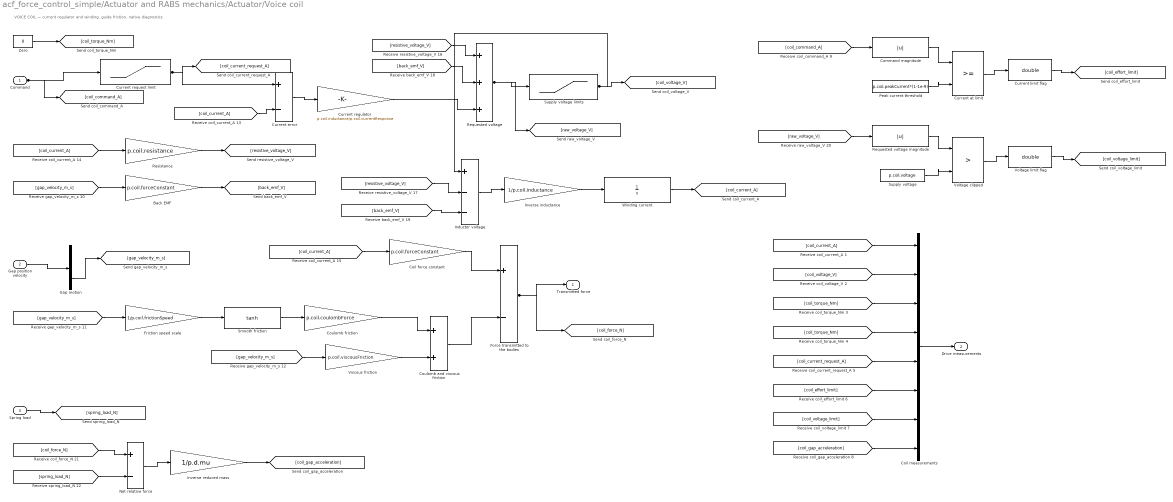
== system acf_force_control_simple/Actuator and RABS mechanics/Actuator/Voice coil ==
  note: VOICE COIL — current regulator and winding, guide friction, native diagnostics
  Command : Inport
  Gap position velocity : Inport  Port=2
  Spring load : Inport  Port=3
  Back EMF : Gain  Gain=p.coil.forceConstant
  Coil force constant : Gain  Gain=p.coil.forceConstant
  Coil measurements : Mux  Inputs=8
  Command magnitude : Abs  SaturateOnIntegerOverflow=off
  Coulomb and viscous friction : Sum
  Coulomb friction : Gain  Gain=p.coil.coulombForce
  Current at limit : RelationalOperator  OutDataTypeStr=boolean  RndMeth=Simplest  InputSameDT=off
  Current error : Sum  Inputs=+-
  Current limit flag : DataTypeConversion  OutDataTypeStr=double  SaturateOnIntegerOverflow=off  RndMeth=Floor
  Current regulator : Gain  Gain=p.coil.inductance/p.coil.currentResponse
  Current request limit : Saturate  UpperLimit=p.coil.peakCurrent  LowerLimit=-p.coil.peakCurrent
  Force transmitted to the bodies : Sum  Inputs=+-
  Friction speed scale : Gain  Gain=1/p.coil.frictionSpeed
  Gap motion : Demux  Outputs=2
  Inductor voltage : Sum  Inputs=+--
  Inverse inductance : Gain  Gain=1/p.coil.inductance
  Inverse reduced mass : Gain  Gain=1/p.d.mu
  Net relative force : Sum  Inputs=+-
  Peak current threshold : Constant  Value=p.coil.peakCurrent*(1-1e-9)
  Requested voltage : Sum  Inputs=+++
  Requested voltage magnitude : Abs  SaturateOnIntegerOverflow=off
  Resistance : Gain  Gain=p.coil.resistance
  Smooth friction : Trigonometry  Operator=tanh
  Supply voltage : Constant  Value=p.coil.voltage
  Supply voltage limits : Saturate  UpperLimit=p.coil.voltage  LowerLimit=-p.coil.voltage
  Viscous friction : Gain  Gain=p.coil.viscousFriction
  Voltage clipped : RelationalOperator  Operator=>  OutDataTypeStr=boolean  RndMeth=Simplest  InputSameDT=off
  Voltage limit flag : DataTypeConversion  OutDataTypeStr=double  SaturateOnIntegerOverflow=off  RndMeth=Floor
  Winding current : Integrator  InitialCondition=p.d.coilHoldCurrent
  Zero : Constant  Value=0
  Transmitted force : Outport
  Drive measurements : Outport  Port=2
  wires:
  Winding current/1 -> [coil_current_A]
  Inductor voltage/1 -> Inverse inductance/1
  [back_emf_V] -> Inductor voltage/3
  Coil force constant/1 -> Force transmitted to the bodies/1
  Requested voltage/1 -> Supply voltage limits/1, [raw_voltage_V]
  Force transmitted to the bodies/1 -> Transmitted force/1, [coil_force_N]
  Current limit flag/1 -> [coil_effort_limit]
  Coulomb friction/1 -> Coulomb and viscous friction/1
  [resistive_voltage_V] -> Requested voltage/1
  [gap_velocity_m_s] -> Viscous friction/1
  [back_emf_V] -> Requested voltage/2
  Smooth friction/1 -> Coulomb friction/1
  Inverse reduced mass/1 -> [coil_gap_acceleration]
  Voltage limit flag/1 -> [coil_voltage_limit]
  Current at limit/1 -> Current limit flag/1
  Current error/1 -> Current regulator/1
  [coil_voltage_V] -> Coil measurements/2
  [coil_effort_limit] -> Coil measurements/6
  Current request limit/1 -> [coil_current_request_A], Current error/1
  [coil_current_A] -> Coil measurements/1
  [gap_velocity_m_s] -> Back EMF/1
  Resistance/1 -> [resistive_voltage_V]
  [coil_force_N] -> Net relative force/1
  [resistive_voltage_V] -> Inductor voltage/2
  [coil_current_A] -> Resistance/1
  Peak current threshold/1 -> Current at limit/2
  Voltage clipped/1 -> Voltage limit flag/1
  Back EMF/1 -> [back_emf_V]
  Spring load/1 -> [spring_load_N]
  [coil_current_A] -> Coil force constant/1
  [gap_velocity_m_s] -> Friction speed scale/1
  Supply voltage limits/1 -> [coil_voltage_V], Inductor voltage/1
  Gap motion/2 -> [gap_velocity_m_s]
  [coil_command_A] -> Command magnitude/1
  Inverse inductance/1 -> Winding current/1
  [coil_torque_Nm] -> Coil measurements/4
  Gap position velocity/1 -> Gap motion/1
  [spring_load_N] -> Net relative force/2
  Command/1 -> [coil_command_A], Current request limit/1
  [coil_voltage_limit] -> Coil measurements/7
  [coil_current_A] -> Current error/2
  Zero/1 -> [coil_torque_Nm]
  Viscous friction/1 -> Coulomb and viscous friction/2
  [coil_torque_Nm] -> Coil measurements/3
  Command magnitude/1 -> Current at limit/1
  [coil_current_request_A] -> Coil measurements/5
  Coil measurements/1 -> Drive measurements/1
  Requested voltage magnitude/1 -> Voltage clipped/1
  [coil_gap_acceleration] -> Coil measurements/8
  [raw_voltage_V] -> Requested voltage magnitude/1
  Net relative force/1 -> Inverse reduced mass/1
  Coulomb and viscous friction/1 -> Force transmitted to the bodies/2
  Supply voltage/1 -> Voltage clipped/2
  Current regulator/1 -> Requested voltage/3
  Friction speed scale/1 -> Smooth friction/1

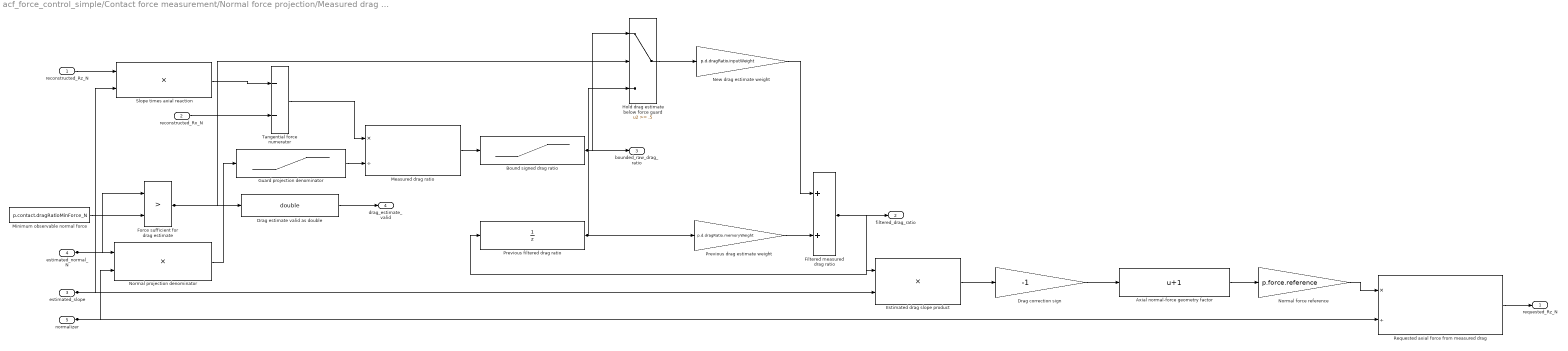
== system acf_force_control_simple/Contact force measurement/Normal force projection/Measured drag geometry ==
  reconstructed_Rz_N : Inport
  reconstructed_Rx_N : Inport  Port=2
  estimated_slope : Inport  Port=3
  estimated_normal_N : Inport  Port=4
  normalizer : Inport  Port=5
  Axial normal-force geometry factor : Bias  Bias=1  SaturateOnIntegerOverflow=off
  Bound signed drag ratio : Saturate  UpperLimit=1  LowerLimit=-1
  Drag correction sign : Gain  Gain=-1
  Drag estimate valid as double : DataTypeConversion  OutDataTypeStr=double  SaturateOnIntegerOverflow=off  RndMeth=Floor
  Estimated drag slope product : Product  Inputs=**
  Filtered measured drag ratio : Sum
  Force sufficient for drag estimate : RelationalOperator  Operator=>  OutDataTypeStr=boolean  RndMeth=Simplest  InputSameDT=off
  Guard projection denominator : Saturate  UpperLimit=inf  LowerLimit=p.contact.dragRatioMinForce_N
  Hold drag estimate below force guard : Switch  Threshold=.5  SaturateOnIntegerOverflow=off  InputSameDT=off
  Measured drag ratio : Product  Inputs=*/
  Minimum observable normal force : Constant  Value=p.contact.dragRatioMinForce_N
  New drag estimate weight : Gain  Gain=p.d.dragRatio.inputWeight
  Normal force reference : Gain  Gain=p.force.reference
  Normal projection denominator : Product  Inputs=**
  Previous drag estimate weight : Gain  Gain=p.d.dragRatio.memoryWeight
  Previous filtered drag ratio : UnitDelay  SampleTime=p.force.sampleTime
  Requested axial force from measured drag : Product  Inputs=*/
  Slope times axial reaction : Product  Inputs=**
  Tangential force numerator : Sum  Inputs=--
  requested_Rz_N : Outport
  filtered_drag_ratio : Outport  Port=2
  bounded_raw_drag_ratio : Outport  Port=3
  drag_estimate_valid : Outport  Port=4
  wires:
  Normal force reference/1 -> Requested axial force from measured drag/1
  Drag correction sign/1 -> Axial normal-force geometry factor/1
  Estimated drag slope product/1 -> Drag correction sign/1
  Filtered measured drag ratio/1 -> Estimated drag slope product/1, filtered_drag_ratio/1, Previous filtered drag ratio/1
  Requested axial force from measured drag/1 -> requested_Rz_N/1
  reconstructed_Rz_N/1 -> Slope times axial reaction/1
  New drag estimate weight/1 -> Filtered measured drag ratio/1
  Previous filtered drag ratio/1 -> Hold drag estimate below force guard/3, Previous drag estimate weight/1
  normalizer/1 -> Normal projection denominator/2, Requested axial force from measured drag/2
  Minimum observable normal force/1 -> Force sufficient for drag estimate/2
  Bound signed drag ratio/1 -> Hold drag estimate below force guard/1, bounded_raw_drag_ratio/1
  estimated_normal_N/1 -> Normal projection denominator/1, Force sufficient for drag estimate/1
  estimated_slope/1 -> Slope times axial reaction/2, Estimated drag slope product/2
  Force sufficient for drag estimate/1 -> Drag estimate valid as double/1, Hold drag estimate below force guard/2
  Slope times axial reaction/1 -> Tangential force numerator/1
  Normal projection denominator/1 -> Guard projection denominator/1
  Drag estimate valid as double/1 -> drag_estimate_valid/1
  reconstructed_Rx_N/1 -> Tangential force numerator/2
  Axial normal-force geometry factor/1 -> Normal force reference/1
  Hold drag estimate below force guard/1 -> New drag estimate weight/1
  Tangential force numerator/1 -> Measured drag ratio/1
  Measured drag ratio/1 -> Bound signed drag ratio/1
  Previous drag estimate weight/1 -> Filtered measured drag ratio/2
  Guard projection denominator/1 -> Measured drag ratio/2

== system acf_force_control_simple/Force controller/Coil PI and PID/Lower spring inverse feedforward ==
  Desired lower load deviation : Sum  Inputs=+-
  Full native inverse log : ToWorkspace  VariableName=lower_inverse_log  SaveFormat=Timeseries  SampleTime=-1
  Known downstream S inertia : Gain  Gain=p.sensor.distalMass_model_kg
  Native audit sampling : ZeroOrderHold  SampleTime=p.sim.step
  Native inverse audit : Mux
  Optional inverse feedforward scale : Gain  Gain=(double(p.inertial.lowerLoadInverse.enabled)*p.inertial.lowerLoadInverse.scale)*double(p.force.feedforwardEnabled)
  Proper identified lower-link inverse : DiscreteTransferFcn  Numerator=p.inertial.lowerLoadInverse.numerator  Denominator=p.inertial.lowerLoadInverse.denominator  InitialStates=zeros(3,1)  SampleTime=p.force.sampleTime
  extra_current_A : Outport
  wires:
  Native inverse audit/1 -> Native audit sampling/1
  Proper identified lower-link inverse/1 -> Optional inverse feedforward scale/1
  Native audit sampling/1 -> Full native inverse log/1
  Desired lower load deviation/1 -> Proper identified lower-link inverse/1, Native inverse audit/3
  [inertial_axial_reference_deviation_N] -> Desired lower load deviation/1, Native inverse audit/1
  Optional inverse feedforward scale/1 -> extra_current_A/1, Native inverse audit/4
  Known downstream S inertia/1 -> Desired lower load deviation/2, Native inverse audit/2
  [measured_S_acceleration_z] -> Known downstream S inertia/1
